simulink model "RetinaGuide_ScreeningWorkflow_Final"  (R2026b)
settings: Solver=VariableStepAuto  StopTime=10
settings Model: Creator=azizn  LastModifiedBy=azizn

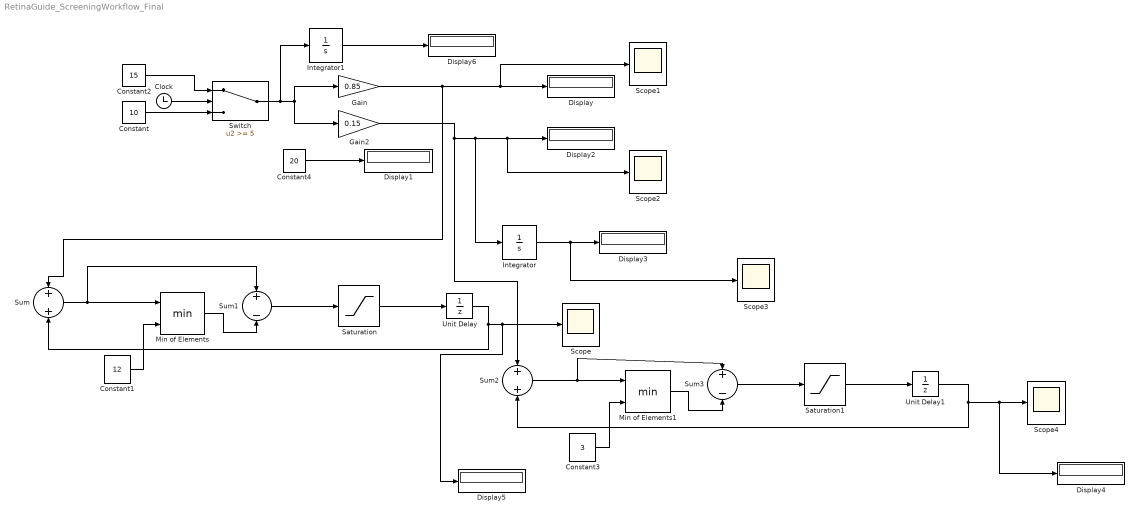
== system RetinaGuide_ScreeningWorkflow_Final ==
  Clock : Clock
  Constant : Constant  Value=10
  Constant1 : Constant  Value=12
  Constant2 : Constant  Value=15
  Constant3 : Constant  Value=3
  Constant4 : Constant  Value=20
  Display{,1..6} (7 alike) : Display
  Gain : Gain  Gain=0.85
  Gain2 : Gain  Gain=0.15
  Integrator : Integrator
  Integrator1 : Integrator
  Min of Elements : MinMax  Inputs=2
  Min of Elements1 : MinMax  Inputs=2
  Saturation : Saturate  UpperLimit=inf  LowerLimit=0
  Saturation1 : Saturate  UpperLimit=inf  LowerLimit=0
  Scope{,1..4} (5 alike) : Scope
      Scope settings: MaximizeAxes=On  ActiveDisplayYMinimum=-12.240690959727669  ActiveDisplayYMaximum=3.1420149338189685
      Scope1 settings: MaximizeAxes=On  ActiveDisplayYMinimum=-376.45397224221705  ActiveDisplayYMaximum=441.94471554227556
      Scope2 settings: MaximizeAxes=On  ActiveDisplayYMinimum=-604.97384104084836  ActiveDisplayYMaximum=938.2389426584424  DataLoggingVariableName=ScopeData2
      Scope3 settings: MaximizeAxes=On  ActiveDisplayYMinimum=0.84507244382960689  ActiveDisplayYMaximum=8.2534628574181816  DataLoggingVariableName=ScopeData3
      Scope4 settings: MaximizeAxes=On  ActiveDisplayYMinimum=-15.034991620496616  ActiveDisplayYMaximum=1.0647288866381537  DataLoggingVariableName=ScopeData4
  Sum : Sum
  Sum1 : Sum  Inputs=+-
  Sum2 : Sum
  Sum3 : Sum  Inputs=+-
  Switch : Switch  Threshold=5  SaturateOnIntegerOverflow=off  InputSameDT=off
  Unit Delay : UnitDelay
  Unit Delay1 : UnitDelay
  wires:
  Constant1/1 -> Min of Elements/2
  Sum1/1 -> Saturation/1
  Saturation/1 -> Unit Delay/1
  Unit Delay/1 -> Sum/2, Display5/1, Scope/1
  Sum/1 -> Sum1/1, Min of Elements/1
  Min of Elements/1 -> Sum1/2
  Constant2/1 -> Switch/1
  Switch/1 -> Integrator1/1, Gain/1, Gain2/1
  Gain2/1 -> Sum2/1, Integrator/1, Scope2/1, Display2/1
  Constant4/1 -> Display1/1
  Clock/1 -> Switch/2
  Constant/1 -> Switch/3
  Gain/1 -> Scope1/1, Display/1, Sum/1
  Integrator/1 -> Scope3/1, Display3/1
  Unit Delay1/1 -> Sum2/2, Display4/1, Scope4/1
  Saturation1/1 -> Unit Delay1/1
  Constant3/1 -> Min of Elements1/2
  Sum2/1 -> Sum3/1, Min of Elements1/1
  Sum3/1 -> Saturation1/1
  Min of Elements1/1 -> Sum3/2
  Integrator1/1 -> Display6/1
